simulink model "example11_2"  (R2021b)
settings: Solver=FixedStepAuto  StartTime=0.0  StopTime=100  FixedStep=0.01  RelTol=1e-3
InitFcn:
  | example11_2_param;
values from neighbouring files (symbols this model uses):
  A = [0 1 0;0 0 1;0 -24 -10]    [example11_2_param.m]
  B = [0 ; 10 ; -80]    [example11_2_param.m]
  C = [1 0 0]    [example11_2_param.m]
  G = [20 ; 76 ; -240]    [example11_2_param.m]
  K = [1.25 1.25 0.19]    [example11_2_param.m]

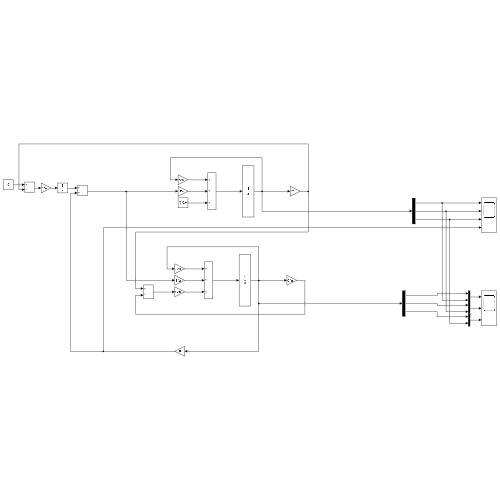
[thumbnail: Simulink's stored preview of the top-level diagram]
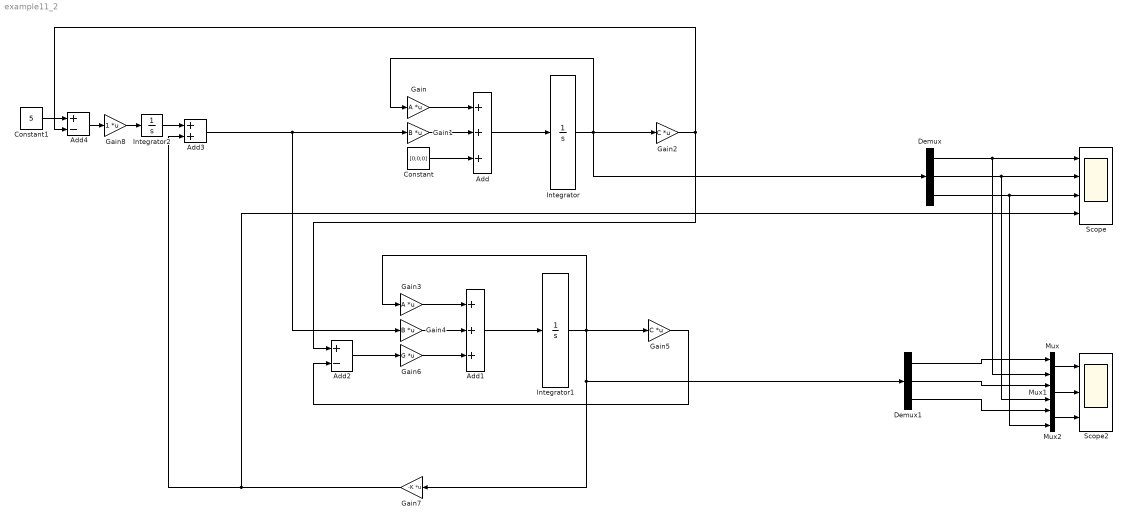
== system example11_2 ==
  Add : Sum  Inputs=+++
  Add1 : Sum  Inputs=+++
  Add2 : Sum  Inputs=+-
  Add3 : Sum
  Add4 : Sum  Inputs=+-
  Constant : Constant  Value=[0;0;0]
  Constant1 : Constant  Value=5
  Demux : Demux  Outputs=3
  Demux1 : Demux  Outputs=3
  Gain : Gain  Gain=A  Multiplication=Matrix(K*u)
  Gain1 : Gain  Gain=B  Multiplication=Matrix(K*u)
  Gain2 : Gain  Gain=C  Multiplication=Matrix(K*u)
  Gain3 : Gain  Gain=A  Multiplication=Matrix(K*u)
  Gain4 : Gain  Gain=B  Multiplication=Matrix(K*u)
  Gain5 : Gain  Gain=C  Multiplication=Matrix(K*u)
  Gain6 : Gain  Gain=G  Multiplication=Matrix(K*u)
  Gain7 : Gain  Gain=-K  Multiplication=Matrix(K*u)
  Gain8 : Gain  Multiplication=Matrix(K*u)
  Integrator : Integrator  InitialCondition=[1;0;0]
  Integrator1 : Integrator  InitialCondition=[0;0;0]
  Integrator2 : Integrator
  Mux : Mux  Inputs=2
  Mux1 : Mux  Inputs=2
  Mux2 : Mux  Inputs=2
  Scope : Scope  NumInputPorts=4
  Scope2 : Scope  NumInputPorts=3
  wires:
  Add/1 -> Integrator/1
  Gain/1 -> Add/1
  Gain1/1 -> Add/2
  Integrator/1 -> Demux/1, Gain2/1, Gain/1
  Integrator1/1 -> Demux1/1, Gain7/1, Gain3/1, Gain5/1
  Gain4/1 -> Add1/2
  Gain3/1 -> Add1/1
  Add1/1 -> Integrator1/1
  Gain2/1 -> Add2/1, Add4/2
  Add2/1 -> Gain6/1
  Gain5/1 -> Add2/2
  Gain6/1 -> Add1/3
  Gain7/1 -> Add3/2, Scope/4
  Demux/1 -> Mux/2, Scope/1
  Demux/2 -> Mux1/2, Scope/2
  Demux/3 -> Mux2/2, Scope/3
  Demux1/1 -> Mux/1
  Demux1/2 -> Mux1/1
  Demux1/3 -> Mux2/1
  Mux/1 -> Scope2/1
  Mux1/1 -> Scope2/2
  Mux2/1 -> Scope2/3
  Constant/1 -> Add/3
  Integrator2/1 -> Add3/1
  Add3/1 -> Gain4/1, Gain1/1
  Constant1/1 -> Add4/1
  Add4/1 -> Gain8/1
  Gain8/1 -> Integrator2/1
